simulink model "TestEncoders"  (R2022b)
settings: Solver=FixedStepAuto  StartTime=0.0  StopTime=inf  RelTol=1e-3  EnableMultiTasking=on
libraries: arduinosensorlib x2
settings Model: ExtModeTrigDuration=2  Creator=miriamfreiriasanjuan  LastModifiedBy=miriamfreiriasanjuan
settings OptimizationCC: EnhancedBackFolding=on  PassReuseOutputArgsAs=Individual arguments  ZeroExternalMemoryAtStartup=off  ZeroInternalMemoryAtStartup=off  MaxStackSize=64  OptimizeBlockOrder=speed  DifferentSizesBufferReuse=on  OptimizationCustomize=off  EfficientTunableParamExpr=on
settings DebuggingCC: ParameterTunabilityLossMsg=error
settings HardwareCC: ProdBitPerInt=16  ProdBitPerPointer=16  ProdBitPerSizeT=16  ProdBitPerPtrDiffT=16  ProdLargestAtomicFloat=None  ProdWordSize=8  ProdHWDeviceType=Atmel->AVR
settings SFSimCC: MATLABDynamicMemAlloc=off
settings RTWCC: Description=Embedded Coder  SystemTargetFile=ert.tlc  HardwareBoard=Arduino Mega 2560  TLCOptions=-aInlineSetEventsForThisBaseRateFcn=TLC_FALSE -aSuppressMultiTaskScheduler=TLC_FALSE -aRateBasedStepFcn=1  TemplateMakefile=ert_default_tmf  Toolchain=Arduino AVR  BuildConfiguration=Faster Runs
settings CodeAppCC: ForceParamTrailComments=on  IgnoreCustomStorageClasses=off  OperatorAnnotations=on  SimulinkDataObjDesc=on  SFDataObjDesc=on  InsertBlockDesc=on
settings ERTTargetCC: SupportContinuousTime=on  SupportVariableSizeSignals=on  ExtModeTransport=3  ExtModeStaticAlloc=on  ExtModeAutomaticAllocSize=off  ExtModeStaticAllocSize=2048  ExtModeMexFile=ext_xcp  ExtModeIntrfLevel=Level2 - Open

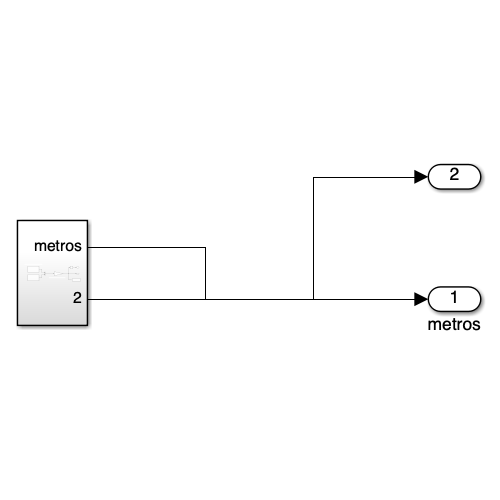
[thumbnail: Simulink's stored preview of the top-level diagram]
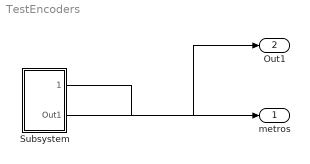
== system TestEncoders ==
  Subsystem : Subsystem
  metros : Outport
  Out1 : Outport  Port=2
  wires:
  Subsystem/1(metros) -> metros/1
  Subsystem/2(Out1) -> Out1/1

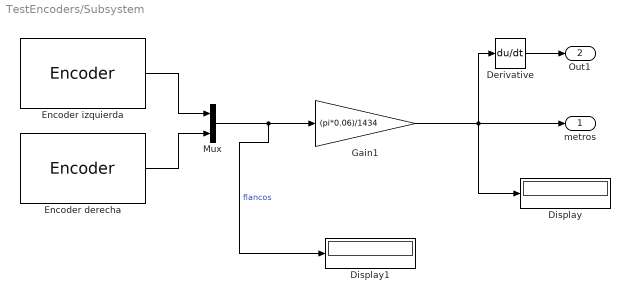
== system TestEncoders/Subsystem ==
  Derivative : Derivative
  Display : Display
  Display1 : Display
  Encoder derecha : arduinosensorlib/Encoder  InputA=2  InputB=3  Mode=No reset  SampleTime=-1
  Encoder izquierda : arduinosensorlib/Encoder  InputA=19  InputB=18  Mode=No reset  SampleTime=-1
  Gain1 : Gain  Gain=(pi*0.06)/1434  ParamDataTypeStr=double  OutDataTypeStr=double
  Mux : Mux  Inputs=2
  metros : Outport
  Out1 : Outport  Port=2
  wires:
  Mux/1 -> Display1/1, Gain1/1  "flancos"
  Encoder izquierda/1 -> Mux/1
  Derivative/1 -> Out1/1
  Encoder derecha/1 -> Mux/2
  Gain1/1 -> metros/1, Display/1, Derivative/1
